simulink model "TP2simu"  (R2022b)
settings: Solver=ode15s  StartTime=0.0  StopTime=60  FixedStep=0.01  RelTol=1e-3
values from neighbouring files (symbols this model uses):
  noise_on = true    [param.m]
  P0 = diag([0.5^2, 0.5^2, (pi/4)^2])    [param.m]
  Q_ekf = diag([q_pos, q_pos, q_alpha])    [param.m]
  R_ekf = diag([sigma_meas^2, sigma_meas^2])    [param.m]
  sigma_meas = 0.01    [param.m]
  u_amp = 0.3    [param.m]
  u_bias = 0.0    (= 0)    [param.m]
  u_freq = 0.1    [param.m]
  Xhat0 = [0.3; 0.7; 0.2]    [param.m]
settings Model: Creator=jdubuc222  LastModifiedBy=jdubuc222

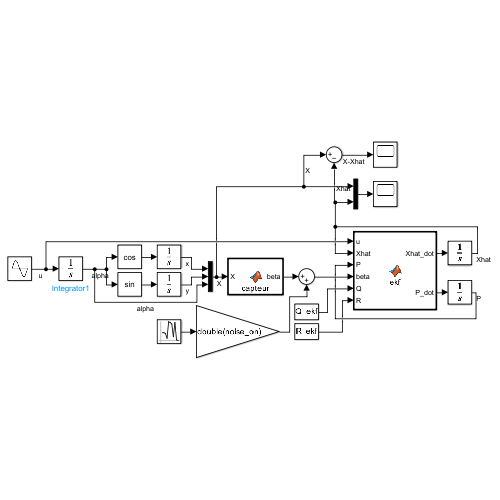
[thumbnail: Simulink's stored preview of the top-level diagram]
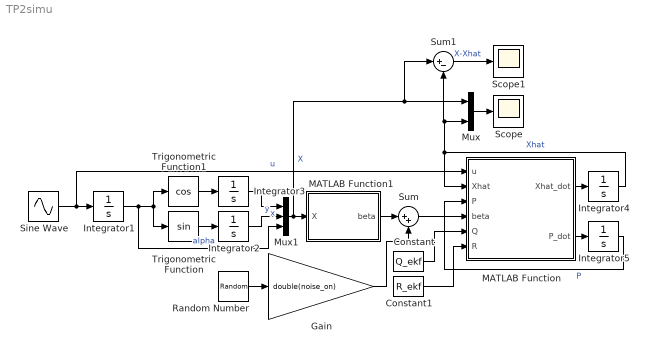
== system TP2simu ==
  Constant : Constant  Value=Q_ekf
  Constant1 : Constant  Value=R_ekf
  Gain : Gain  Gain=double(noise_on)
  Integrator1 : Integrator
  Integrator2 : Integrator
  Integrator3 : Integrator
  Integrator4 : Integrator  InitialCondition=Xhat0
  Integrator5 : Integrator  InitialCondition=P0
  MATLAB Function : MATLAB Function  TreatAsAtomicUnit=on
  MATLAB Function1 : MATLAB Function  TreatAsAtomicUnit=on
  Mux : Mux  Inputs=2
  Mux1 : Mux  Inputs=3
  Random Number : RandomNumber  Variance=sigma_meas^2  Seed=1  SampleTime=0.01
  Scope : Scope
  Scope1 : Scope
  Sine Wave : Sin  Amplitude=u_amp  Bias=u_bias  Frequency=2*pi*u_freq  SampleTime=0
  Sum : Sum  Inputs=|++
  Sum1 : Sum  Inputs=|+-
  Trigonometric Function : Trigonometry
  Trigonometric Function1 : Trigonometry  Operator=cos
  wires:
  Sine Wave/1 -> MATLAB Function/1(u), Integrator1/1  "u"
  Mux/1 -> Scope/1
  Integrator1/1 -> Mux1/3, Trigonometric Function1/1, Trigonometric Function/1  "alpha"
  Trigonometric Function/1 -> Integrator2/1
  Trigonometric Function1/1 -> Integrator3/1
  Integrator2/1 -> Mux1/2  "y"
  Integrator3/1 -> Mux1/1  "x"
  MATLAB Function/1(Xhat_dot) -> Integrator4/1
  MATLAB Function/2(P_dot) -> Integrator5/1
  Integrator4/1 -> MATLAB Function/2(Xhat), Mux/2, Sum1/2  "Xhat"
  Integrator5/1 -> MATLAB Function/3(P)  "P"
  Mux1/1 -> Mux/1, Sum1/1, MATLAB Function1/1(X)  "X"
  Constant/1 -> MATLAB Function/5(Q)
  Constant1/1 -> MATLAB Function/6(R)
  Random Number/1 -> Gain/1
  Gain/1 -> Sum/2
  Sum1/1 -> Scope1/1  "X-Xhat"
  MATLAB Function1/1(beta) -> Sum/1
  Sum/1 -> MATLAB Function/4(beta)

== matlab function TP2simu/MATLAB Function1 ==
  data: X input; beta output
function beta = capteur(X)

x = X(1); y = X(2); alpha = X(3);

% Représentants locaux continus (pas de modulo)

beta_A = pi + atan2(y, x) - alpha;

beta_B = pi + atan2(y, x - 1) - alpha;

beta = [beta_A; beta_B];

end

== matlab function TP2simu/MATLAB Function ==
  data: u input; Xhat_dot output; Xhat input; P input; beta input; Q input; R input; P_dot output
function [Xhat_dot, P_dot] = ekf(u, Xhat, P, beta, Q, R)
    % EKF Continu pour le modèle de Dubins
    x = Xhat(1); 
    y = Xhat(2); 
    alpha = Xhat(3);

    % --- Modèle dynamique f(X, u) ---
    f_x = [cos(alpha); 
           sin(alpha); 
           u];

    % --- Jacobienne de la dynamique (F) ---
    F = [0, 0, -sin(alpha);
         0, 0,  cos(alpha);
         0, 0,  0];

    % --- Modèle de mesure h(X) ---
    h_x = [pi + atan2(y, x)     - alpha;
           pi + atan2(y, x - 1) - alpha];

    % --- Jacobienne de la mesure (H) ---
    % Ajout de 1e-12 pour éviter la division par zéro (singularité)
    d1 = x^2 + y^2 + 1e-12;
    d2 = (x - 1)^2 + y^2 + 1e-12;
    
    H = [ -y/d1,  x/d1,     -1;
          -y/d2, (x - 1)/d2, -1 ];

    % --- Gain de Kalman (K) ---
    K = (P * H') / R;

    % --- Calcul de l'innovation robuste ---
    % On force la différence d'angle à rester entre -pi et +pi
    erreur_brute = beta - h_x;
    innovation = atan2(sin(erreur_brute), cos(erreur_brute));

    % --- Équation différentielle de l'état estimé ---
    Xhat_dot = f_x + K * innovation;

    % --- Équation différentielle de Riccati pour la covariance (P) ---
    P_dot = F*P + P*F' + Q - K*H*P;
    
    % Force la symétrie pour empêcher la dérive numérique
    P_dot = (P_dot + P_dot') / 2;
end
